simulink model "Cannon_Fire"  (R2025b)
settings: Solver=ode8  StartTime=0.0  StopTime=25  FixedStep=0.01  RelTol=1e-4
settings Model: Creator=bala4krish  LastModifiedBy=MehrSystem
settings SolverCC: AlgebraicLoopSolver=TrustRegion
settings DebuggingCC: UnconnectedInputMsg=warning  UnconnectedOutputMsg=warning  UnconnectedLineMsg=warning
settings ModelReferenceCC: EnableRefExpFcnMdlSchedulingChecks=on
settings RTWCC: GPUComputeCapability=3.5

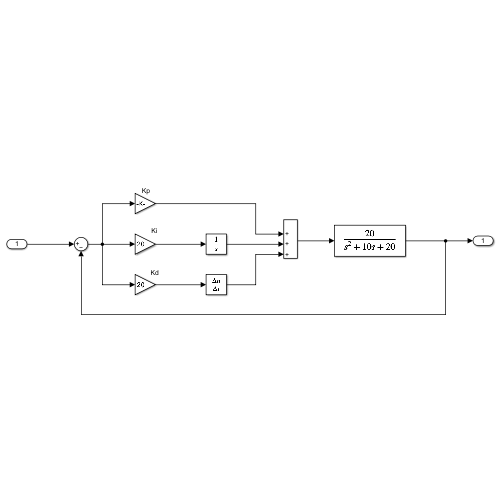
[thumbnail: Simulink's stored preview of the top-level diagram]
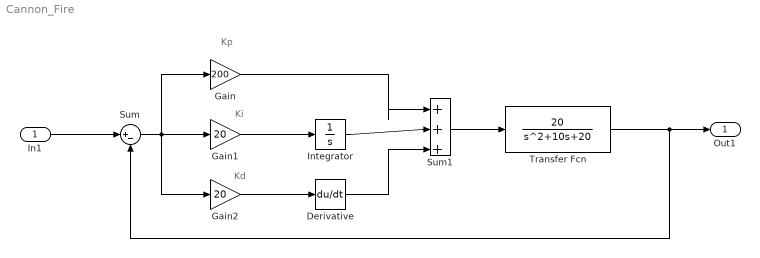
== system Cannon_Fire ==
  note: Kd
  note: Ki
  note: Kp
  In1 : Inport
  Derivative : Derivative
  Gain : Gain  Gain=200
  Gain1 : Gain  Gain=20
  Gain2 : Gain  Gain=20
  Integrator : Integrator
  Sum : Sum  Inputs=|+-
  Sum1 : Sum  Inputs=|+++
  Transfer Fcn : TransferFcn  Numerator=[20]  Denominator=[1 10 20]
  Out1 : Outport
  wires:
  In1/1 -> Sum/1
  Sum/1 -> Gain2/1, Gain/1, Gain1/1
  Gain1/1 -> Integrator/1
  Sum1/1 -> Transfer Fcn/1
  Integrator/1 -> Sum1/2
  Gain/1 -> Sum1/1
  Gain2/1 -> Derivative/1
  Derivative/1 -> Sum1/3
  Transfer Fcn/1 -> Out1/1, Sum/2
